simulink model "DBVF_2027"  (R2026b)
settings: Solver=ode4  StopTime=200  FixedStep=0.01
values from neighbouring files (symbols this model uses):
  Ah = 10    [model_workspace.m]
  all_written = 8191    [model_workspace.m]
  deg_to_cdeg = 100    [model_workspace.m]
  degE7 = 1.0E+7    (= 10000000)    [model_workspace.m]
  ground_elevation_m = 221    [model_workspace.m]
  I_0 = 0.31    [model_workspace.m]
  I_max = 100    [model_workspace.m]
  J_m = 8.6200e-04 * 1.5    (= 0.001293)    [model_workspace.m]
  K_e = 0.03080418253    [model_workspace.m]
  K_t = 0.03080418253    [model_workspace.m]
  K_u = 1    [model_workspace.m]
  m_to_cm = 100    [model_workspace.m]
  m_to_mm = 1000    [model_workspace.m]
  mps2_to_mG = 101.97    [model_workspace.m]
  n_cells = 6    [model_workspace.m]
  Pa_to_hPa = 0.01    [model_workspace.m]
  R_batt = 6*10e-4    (= 0.006)    [model_workspace.m]
  R_m = 0.17    [model_workspace.m]
  reference_location = [36.2071 -96.0102 221.3415]    [model_workspace.m]
  rho_kgpm3 = 1.225    [model_workspace.m]
  s_to_us = 1.0E+6    (= 1000000)    [model_workspace.m]
  timestep = 0.005    [model_workspace.m]
  uT_to_gauss = 0.01    [model_workspace.m]
undefined symbols (not defined in the file or in its folder): fractalcoef, Payload
libraries: uavmavlinklib x10, aerolibatmos2 x2, aerolibutil x2, simulink x2, aerolibasang x1, aerolibconvert2 x1, mspsensorlib x1, sharedtransform x1, sensorgpslib x1
settings Model: Creator=Teama  LastModifiedBy=Teama

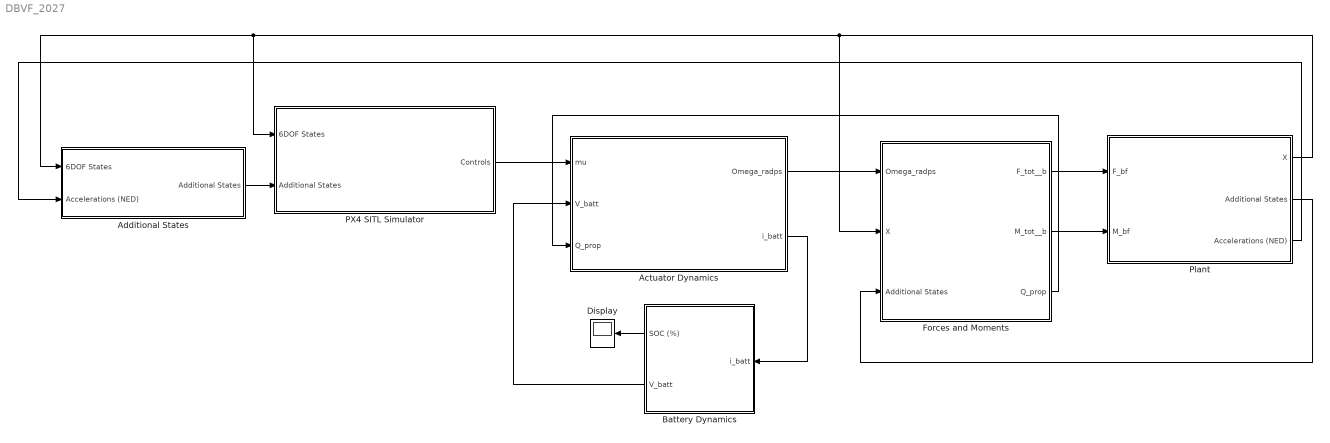
== system DBVF_2027 ==
  Actuator Dynamics : Subsystem
  Additional States : Subsystem
  Battery Dynamics : Subsystem
  Display : Display
  Forces and Moments : Subsystem
  PX4 SITL Simulator : Subsystem
  Plant : Subsystem
  wires:
  Actuator Dynamics/1(Omega_radps) -> Forces and Moments/1(Omega_radps)
  Actuator Dynamics/2(i_batt) -> Battery Dynamics/1(i_batt)
  Battery Dynamics/2(V_batt) -> Actuator Dynamics/2(V_batt)
  Forces and Moments/3(Q_prop) -> Actuator Dynamics/3(Q_prop)
  Additional States/1(Additional States) -> PX4 SITL Simulator/2(Additional States)
  PX4 SITL Simulator/1(Controls) -> Actuator Dynamics/1(mu)
  Battery Dynamics/1(SOC (%)) -> Display/1
  Plant/1(X) -> Forces and Moments/2(X), PX4 SITL Simulator/1(6DOF States), Additional States/1(6DOF States)
  Forces and Moments/1(F_tot__b) -> Plant/1(F_bf)
  Forces and Moments/2(M_tot__b) -> Plant/2(M_bf)
  Plant/2(Additional States) -> Forces and Moments/3(Additional States)
  Plant/3(Accelerations (NED)) -> Additional States/2(Accelerations (NED))

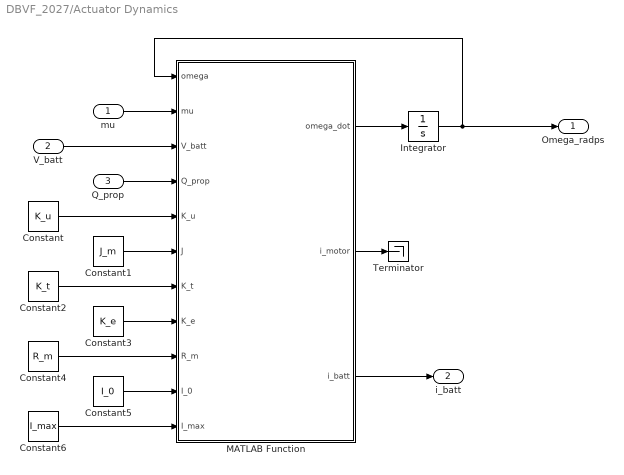
== system DBVF_2027/Actuator Dynamics ==
  mu : Inport
  V_batt : Inport  Port=2
  Q_prop : Inport  Port=3
  Constant : Constant  Value=K_u
  Constant1 : Constant  Value=J_m
  Constant2 : Constant  Value=K_t
  Constant3 : Constant  Value=K_e
  Constant4 : Constant  Value=R_m
  Constant5 : Constant  Value=I_0
  Constant6 : Constant  Value=I_max
  Integrator : Integrator
  MATLAB Function : MATLAB Function  TreatAsAtomicUnit=on
  Terminator : Terminator
  Omega_radps : Outport
  i_batt : Outport  Port=2
  wires:
  mu/1 -> MATLAB Function/2(mu)
  MATLAB Function/1(omega_dot) -> Integrator/1
  Integrator/1 -> MATLAB Function/1(omega), Omega_radps/1
  V_batt/1 -> MATLAB Function/3(V_batt)
  Q_prop/1 -> MATLAB Function/4(Q_prop)
  MATLAB Function/2(i_motor) -> Terminator/1
  MATLAB Function/3(i_batt) -> i_batt/1
  Constant/1 -> MATLAB Function/5(K_u)
  Constant1/1 -> MATLAB Function/6(J)
  Constant2/1 -> MATLAB Function/7(K_t)
  Constant3/1 -> MATLAB Function/8(K_e)
  Constant4/1 -> MATLAB Function/9(R_m)
  Constant5/1 -> MATLAB Function/10(I_0)
  Constant6/1 -> MATLAB Function/11(I_max)

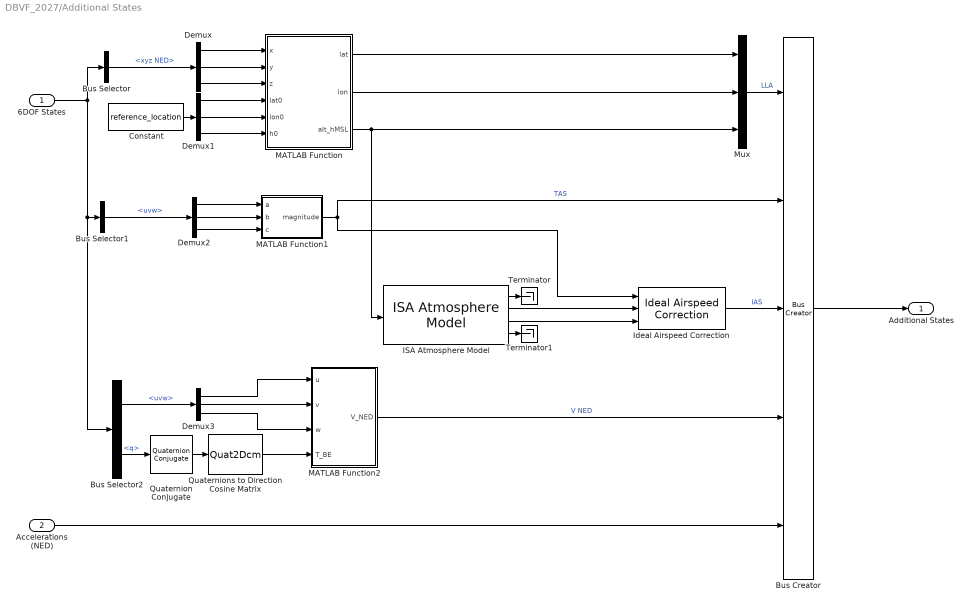
== system DBVF_2027/Additional States ==
  6DOF States : Inport
  Accelerations (NED) : Inport  Port=2
  Bus Creator : BusCreator  Inputs=5
  Bus Selector : BusSelector  OutputSignals=xyz NED
  Bus Selector1 : BusSelector  OutputSignals=uvw
  Bus Selector2 : BusSelector  OutputSignals=uvw,q
  Constant : Constant  Value=reference_location
  Demux{,1..3} (4 alike) : Demux  Outputs=3
  ISA Atmosphere Model : aerolibatmos2/ISA Atmosphere Model  useExtended=off  action=None  custom=off  viscosityOut=off  g=9.80665  gamma=1.4  R=287.0531  L=0.0065  h_trop=11000  h_strat=20000  rho0=1.225  P0=101325  T0=288.15  h0=0  S=110.4  Tref=273.15  muref=1.716e-5
  Ideal Airspeed Correction : aerolibasang/Ideal Airspeed Correction  units=Metric (MKS)  vel_in=TAS  vel_out_tas=CAS  vel_out_eas=TAS  vel_out_cas=TAS  method=Table Lookup  SubOnly=off  action=None
  MATLAB Function : MATLAB Function  TreatAsAtomicUnit=on
  MATLAB Function1 : MATLAB Function  TreatAsAtomicUnit=on
  MATLAB Function2 : MATLAB Function  TreatAsAtomicUnit=on
  Mux : Mux  Inputs=3
  Quaternion Conjugate : aerolibutil/Quaternion Conjugate
  Quaternions to Direction Cosine Matrix : Quat2Dcm
  Terminator : Terminator
  Terminator1 : Terminator
  Additional States : Outport
  wires:
  Bus Creator/1 -> Additional States/1
  6DOF States/1 -> Bus Selector2/1, Bus Selector1/1, Bus Selector/1
  Bus Selector/1 -> Demux/1  "<xyz NED>"
  MATLAB Function/1(lat) -> Mux/1
  MATLAB Function/2(lon) -> Mux/2
  MATLAB Function/3(alt_hMSL) -> Mux/3, ISA Atmosphere Model/1
  Mux/1 -> Bus Creator/1  "LLA"
  Demux/1 -> MATLAB Function/1(x)
  Demux/2 -> MATLAB Function/2(y)
  Demux/3 -> MATLAB Function/3(z)
  Constant/1 -> Demux1/1
  Demux1/1 -> MATLAB Function/4(lat0)
  Demux1/2 -> MATLAB Function/5(lon0)
  Demux1/3 -> MATLAB Function/6(h0)
  Ideal Airspeed Correction/1 -> Bus Creator/3  "IAS"
  Bus Selector1/1 -> Demux2/1  "<uvw>"
  Demux2/1 -> MATLAB Function1/1(a)
  Demux2/2 -> MATLAB Function1/2(b)
  Demux2/3 -> MATLAB Function1/3(c)
  MATLAB Function1/1(magnitude) -> Ideal Airspeed Correction/1, Bus Creator/2  "TAS"
  ISA Atmosphere Model/3 -> Ideal Airspeed Correction/3
  ISA Atmosphere Model/2 -> Ideal Airspeed Correction/2
  ISA Atmosphere Model/1 -> Terminator/1
  ISA Atmosphere Model/4 -> Terminator1/1
  Quaternions to Direction Cosine Matrix/1 -> MATLAB Function2/4(T_BE)
  Bus Selector2/1 -> Demux3/1  "<uvw>"
  Bus Selector2/2 -> Quaternion Conjugate/1  "<q>"
  Demux3/1 -> MATLAB Function2/1(u)
  Demux3/2 -> MATLAB Function2/2(v)
  Demux3/3 -> MATLAB Function2/3(w)
  MATLAB Function2/1(V_NED) -> Bus Creator/4  "V NED"
  Quaternion Conjugate/1 -> Quaternions to Direction Cosine Matrix/1
  Accelerations (NED)/1 -> Bus Creator/5

== system DBVF_2027/Battery Dynamics ==
  i_batt : Inport
  Constant : Constant  Value=Ah
  Constant1 : Constant  Value=R_batt
  Gain : Gain  Gain=n_cells
  Gain1 : Gain  Gain=100
  Integrator : Integrator
  LiPo Discharge Curve : Lookup_n-D  NumberOfTableDimensions=1  BreakpointsForDimension1="[0    0.05  0.10  0.20  0.30  0.40  0.50  0.60  0.70  0.80  0.90  1.00]"  Table="[3.20 3.45  3.55  3.65  3.70  3.74  3.77  3.80  3.84  3.90  4.00  4.20]"  InternalRulePriority=Speed  RndMeth=Simplest
  battery dynamics wrapper : MATLAB Function  TreatAsAtomicUnit=on
  SOC (%) : Outport
  V_batt : Outport  Port=2
  wires:
  i_batt/1 -> battery dynamics wrapper/1(I_batt_in)
  battery dynamics wrapper/1(SOC_dot) -> Integrator/1
  Integrator/1 -> Gain1/1, LiPo Discharge Curve/1
  LiPo Discharge Curve/1 -> Gain/1
  Gain/1 -> battery dynamics wrapper/2(V_OC)
  battery dynamics wrapper/2(V_batt) -> V_batt/1
  Gain1/1 -> SOC (%)/1
  Constant/1 -> battery dynamics wrapper/4(Ah)
  Constant1/1 -> battery dynamics wrapper/3(R_batt)

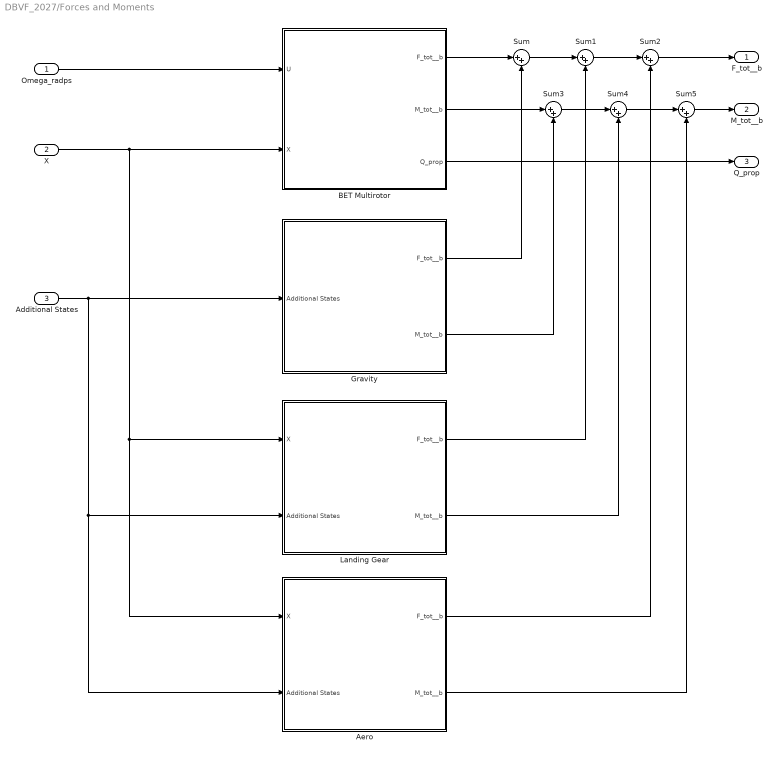
== system DBVF_2027/Forces and Moments ==
  Omega_radps : Inport
  X : Inport  Port=2
  Additional States : Inport  Port=3
  Aero : Subsystem
  BET Multirotor : Subsystem
  Gravity : Subsystem
  Landing Gear : Subsystem
  Sum{,1..5} (6 alike) : Sum  Inputs=|++
  F_tot__b : Outport
  M_tot__b : Outport  Port=2
  Q_prop : Outport  Port=3
  wires:
  Omega_radps/1 -> BET Multirotor/1(U)
  X/1 -> Landing Gear/1(X), Aero/1(X), BET Multirotor/2(X)
  Additional States/1 -> Landing Gear/2(Additional States), Aero/2(Additional States), Gravity/1(Additional States)
  BET Multirotor/1(F_tot__b) -> Sum/1
  Gravity/1(F_tot__b) -> Sum/2
  Sum/1 -> Sum1/1
  Aero/1(F_tot__b) -> Sum2/2
  Sum1/1 -> Sum2/1
  Sum2/1 -> F_tot__b/1
  BET Multirotor/2(M_tot__b) -> Sum3/1
  Gravity/2(M_tot__b) -> Sum3/2
  Sum3/1 -> Sum4/1
  Sum5/1 -> M_tot__b/1
  Sum4/1 -> Sum5/1
  Aero/2(M_tot__b) -> Sum5/2
  BET Multirotor/3(Q_prop) -> Q_prop/1
  Landing Gear/1(F_tot__b) -> Sum1/2
  Landing Gear/2(M_tot__b) -> Sum4/2

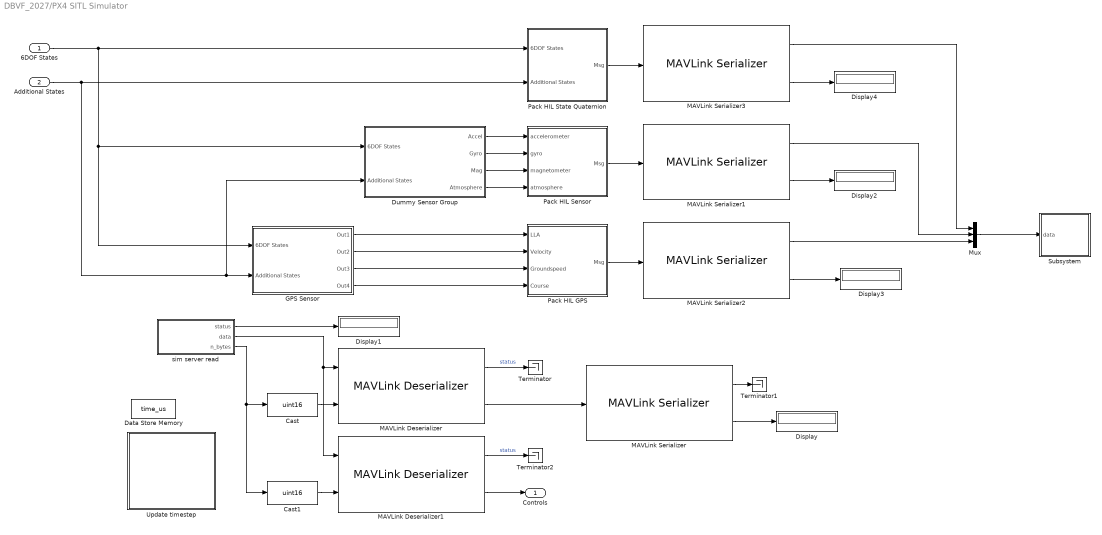
== system DBVF_2027/PX4 SITL Simulator ==
  6DOF States : Inport
  Additional States : Inport  Port=2
  Cast : DataTypeConversion  OutDataTypeStr=uint16  SaturateOnIntegerOverflow=off  RndMeth=Floor
  Cast1 : DataTypeConversion  OutDataTypeStr=uint16  SaturateOnIntegerOverflow=off  RndMeth=Floor
  Data Store Memory : DataStoreMemory  DataStoreName=time_us  WriteAfterWriteMsg=warning  ShowAdditionalParam=off  OutDataTypeStr=uint64
  Display{,1..4} (5 alike) : Display
  Dummy Sensor Group : Subsystem
  GPS Sensor : Subsystem
  MAVLink Deserializer : uavmavlinklib/MAVLink Deserializer  dialectSource=Select from standard MAVLink dialects  dialect=common.xml  dialectCustom=common.xml  version=2  messageType=HEARTBEAT  inputDataLength=on  SystemIDFilter=off  systemID=1  ComponentIDFilter=off  componentID=1  queueMsg=off  queueMsgSize=50  dropNum=off
  MAVLink Deserializer1 : uavmavlinklib/MAVLink Deserializer  dialectSource=Select from standard MAVLink dialects  dialect=common.xml  dialectCustom=common.xml  version=2  messageType=HIL_ACTUATOR_CONTROLS  inputDataLength=on  SystemIDFilter=off  systemID=1  ComponentIDFilter=off  componentID=1  queueMsg=off  queueMsgSize=50  dropNum=off
  MAVLink Serializer : uavmavlinklib/MAVLink Serializer  dialectSource=Select from standard MAVLink dialects  dialect=common.xml  dialectCustom=common.xml  version=2  messageType=HEARTBEAT
  MAVLink Serializer1 : uavmavlinklib/MAVLink Serializer  dialectSource=Select from standard MAVLink dialects  dialect=common.xml  dialectCustom=common.xml  version=2  messageType=HIL_SENSOR
  MAVLink Serializer2 : uavmavlinklib/MAVLink Serializer  dialectSource=Select from standard MAVLink dialects  dialect=common.xml  dialectCustom=common.xml  version=2  messageType=HIL_GPS
  MAVLink Serializer3 : uavmavlinklib/MAVLink Serializer  dialectSource=Select from standard MAVLink dialects  dialect=common.xml  dialectCustom=common.xml  version=2  messageType=HIL_STATE_QUATERNION
  Mux : Mux  Inputs=3
  Pack HIL GPS : Subsystem
  Pack HIL Sensor : Subsystem
  Pack HIL State Quaternion : Subsystem
  Subsystem : Subsystem
  Terminator : Terminator
  Terminator1 : Terminator
  Terminator2 : Terminator
  Update timestep : Subsystem
  sim server read : MATLAB Function  TreatAsAtomicUnit=on
  Controls : Outport
  wires:
  sim server read/1(status) -> Display1/1
  MAVLink Serializer/1 -> Terminator1/1
  MAVLink Serializer3/1 -> Mux/1
  MAVLink Serializer3/2 -> Display4/1
  sim server read/2(data) -> MAVLink Deserializer1/1, MAVLink Deserializer/1
  Dummy Sensor Group/1(Accel) -> Pack HIL Sensor/1(accelerometer)
  Dummy Sensor Group/2(Gyro) -> Pack HIL Sensor/2(gyro)
  Dummy Sensor Group/4(Atmosphere) -> Pack HIL Sensor/4(atmosphere)
  Pack HIL State Quaternion/1(Msg) -> MAVLink Serializer3/1
  Dummy Sensor Group/3(Mag) -> Pack HIL Sensor/3(magnetometer)
  MAVLink Serializer1/1 -> Mux/2
  Additional States/1 -> Dummy Sensor Group/2(Additional States), GPS Sensor/2(Additional States), Pack HIL State Quaternion/2(Additional States)
  MAVLink Serializer2/2 -> Display3/1
  Pack HIL Sensor/1(Msg) -> MAVLink Serializer1/1
  MAVLink Serializer1/2 -> Display2/1
  MAVLink Serializer2/1 -> Mux/3
  MAVLink Serializer/2 -> Display/1
  Pack HIL GPS/1(Msg) -> MAVLink Serializer2/1
  MAVLink Deserializer/1 -> Terminator/1  "status"
  MAVLink Deserializer/2 -> MAVLink Serializer/1
  6DOF States/1 -> GPS Sensor/1(6DOF States), Dummy Sensor Group/1(6DOF States), Pack HIL State Quaternion/1(6DOF States)
  MAVLink Deserializer1/1 -> Terminator2/1  "status"
  MAVLink Deserializer1/2 -> Controls/1
  Mux/1 -> Subsystem/1(data)
  GPS Sensor/1(Out1) -> Pack HIL GPS/1(LLA)
  GPS Sensor/2(Out2) -> Pack HIL GPS/2(Velocity)
  GPS Sensor/3(Out3) -> Pack HIL GPS/3(Groundspeed)
  GPS Sensor/4(Out4) -> Pack HIL GPS/4(Course)
  sim server read/3(n_bytes) -> Cast/1, Cast1/1
  Cast/1 -> MAVLink Deserializer/2
  Cast1/1 -> MAVLink Deserializer1/2

== system DBVF_2027/Plant ==
  F_bf : Inport
  M_bf : Inport  Port=2
  6DOF (Quaternion) : EOM6DOFBodyQuat  xme_0=[0 0 -ground_elevation_m]  mass_0=m_kg  inertia=I_kgm2  mass_flag=on
  A_bf to A_NED : Subsystem
  Bus Creator : BusCreator  Inputs=4
  Bus Creator1 : BusCreator  Inputs=4
  Terminator : Terminator
  X : Outport
  Additional States : Outport  Port=2
  Accelerations (NED) : Outport  Port=3
  wires:
  6DOF (Quaternion)/5 -> A_bf to A_NED/3(DCM_be), Bus Creator1/2  "DCM_be"
  6DOF (Quaternion)/1 -> Bus Creator1/1  "V_e"
  6DOF (Quaternion)/3 -> Terminator/1
  6DOF (Quaternion)/2 -> Bus Creator/1  "X_e"
  M_bf/1 -> 6DOF (Quaternion)/2
  6DOF (Quaternion)/7 -> Bus Creator/3  "Omega_b"
  6DOF (Quaternion)/6 -> Bus Creator/2  "V_b"
  6DOF (Quaternion)/4 -> Bus Creator/4  "q"
  F_bf/1 -> A_bf to A_NED/1(F_bf), 6DOF (Quaternion)/1
  Bus Creator/1 -> X/1
  Bus Creator1/1 -> Additional States/1
  6DOF (Quaternion)/8 -> A_bf to A_NED/2(m), Bus Creator1/3  "m"
  A_bf to A_NED/1(Accelerations (NED)) -> Accelerations (NED)/1
  6DOF (Quaternion)/9 -> Bus Creator1/4  "I"

== system DBVF_2027/Forces and Moments/Aero ==
  X : Inport
  Additional States : Inport  Port=2
  F_tot__b : Outport
  M_tot__b : Outport  Port=2
  wires:
  ? -> F_tot__b/1
  ? -> M_tot__b/1

== system DBVF_2027/Forces and Moments/BET Multirotor ==
  U : Inport
  X : Inport  Port=2
  Constant : Constant  Value=rho_kgpm3  VectorParams1D=off
  Multirotor : Multirotor  modelMode=With flap effects  CTCQMode=Compute using BEMT
  F_tot__b : Outport
  M_tot__b : Outport  Port=2
  Q_prop : Outport  Port=3
  wires:
  Multirotor/2 -> M_tot__b/1
  U/1 -> Multirotor/1
  X/1 -> ?
  Multirotor/1 -> F_tot__b/1
  Constant/1 -> Multirotor/2

== system DBVF_2027/Forces and Moments/Gravity ==
  Additional States : Inport
  Bus Selector : BusSelector  OutputSignals=m,DCM_be
  MATLAB Function : MATLAB Function  TreatAsAtomicUnit=on
  F_tot__b : Outport
  M_tot__b : Outport  Port=2
  wires:
  Bus Selector/2 -> MATLAB Function/2(DCM_be)  "<DCM_be>"
  Bus Selector/1 -> MATLAB Function/1(m)  "<m>"
  Additional States/1 -> Bus Selector/1
  MATLAB Function/1(F_tot__b) -> F_tot__b/1
  MATLAB Function/2(M_tot__b) -> M_tot__b/1

== system DBVF_2027/Forces and Moments/Landing Gear ==
  X : Inport
  Additional States : Inport  Port=2
  Bus Selector : BusSelector  OutputSignals=DCM_be,m
  Constant : Constant  Value=reference_location(3)
  Landing Gear Subsystem : Subsystem  ReferencedSubsystem=Landing_Gear_Subsystem
  F_tot__b : Outport
  M_tot__b : Outport  Port=2
  wires:
  X/1 -> Landing Gear Subsystem/1
  Landing Gear Subsystem/1 -> F_tot__b/1
  Landing Gear Subsystem/2 -> M_tot__b/1
  Additional States/1 -> Bus Selector/1
  Bus Selector/1 -> Landing Gear Subsystem/2  "<DCM_be>"
  Bus Selector/2 -> Landing Gear Subsystem/4  "<m>"
  Constant/1 -> Landing Gear Subsystem/3

== system DBVF_2027/PX4 SITL Simulator/Dummy Sensor Group ==
  6DOF States : Inport
  Additional States : Inport  Port=2
  Dummy Barometer Data : Subsystem
  Dummy IMU Data : Subsystem
  Accel : Outport
  Gyro : Outport  Port=2
  Mag : Outport  Port=3
  Atmosphere : Outport  Port=4
  wires:
  Dummy IMU Data/1(Accel) -> Accel/1
  Dummy IMU Data/2(Gyro) -> Gyro/1
  Dummy IMU Data/3(Mag) -> Mag/1
  Dummy Barometer Data/1(Out1) -> Atmosphere/1
  6DOF States/1 -> Dummy IMU Data/2(6DOF States)
  Additional States/1 -> Dummy IMU Data/1(Additional States), Dummy Barometer Data/1(Additional States)

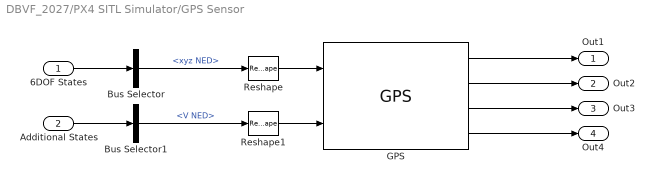
== system DBVF_2027/PX4 SITL Simulator/GPS Sensor ==
  6DOF States : Inport
  Additional States : Inport  Port=2
  Bus Selector : BusSelector  OutputSignals=xyz NED
  Bus Selector1 : BusSelector  OutputSignals=V NED
  GPS : sensorgpslib/GPS  DispRefFrame=NED  PositionInputFormat=Local  ReferenceLocation=reference_location  HorizontalPositionAccuracy=0.01  VerticalPositionAccuracy=0.01  VelocityAccuracy=0.01  DecayFactor=0.99  SeedDouble=67  SimulateUsing=Interpreted execution
      settings: LibrarySourceBlock=mspsensorlib/GPS
  Reshape : Reshape  OutputDimensionality=Row vector (2-D)
  Reshape1 : Reshape  OutputDimensionality=Row vector (2-D)
  Out1 : Outport
  Out2 : Outport  Port=2
  Out3 : Outport  Port=3
  Out4 : Outport  Port=4
  wires:
  Reshape/1 -> GPS/1
  GPS/1 -> Out1/1
  Reshape1/1 -> GPS/2
  Bus Selector/1 -> Reshape/1  "<xyz NED>"
  Bus Selector1/1 -> Reshape1/1  "<V NED>"
  GPS/4 -> Out4/1
  GPS/3 -> Out3/1
  GPS/2 -> Out2/1
  6DOF States/1 -> Bus Selector/1
  Additional States/1 -> Bus Selector1/1

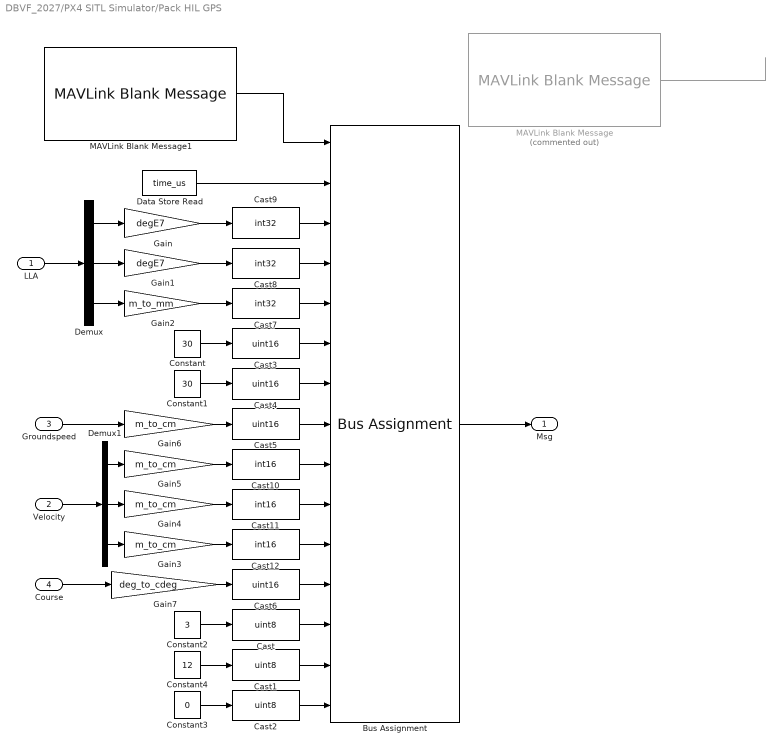
== system DBVF_2027/PX4 SITL Simulator/Pack HIL GPS ==
  LLA : Inport
  Velocity : Inport  Port=2
  Groundspeed : Inport  Port=3
  Course : Inport  Port=4
  Bus Assignment : BusAssignment  AssignedSignals=Payload.time_usec,Payload.lat,Payload.lon,Payload.alt,Payload.eph,Payload.epv,Payload.vel,Payload.vn,Payload.ve,Payload.vd,Payload.cog,Payload.fix_type,Payload.satellites_visible,Payload.id
  Cast : DataTypeConversion  OutDataTypeStr=uint8  SaturateOnIntegerOverflow=off  RndMeth=Floor
  Cast1 : DataTypeConversion  OutDataTypeStr=uint8  SaturateOnIntegerOverflow=off  RndMeth=Floor
  Cast10 : DataTypeConversion  OutDataTypeStr=int16  SaturateOnIntegerOverflow=off  RndMeth=Floor
  Cast11 : DataTypeConversion  OutDataTypeStr=int16  SaturateOnIntegerOverflow=off  RndMeth=Floor
  Cast12 : DataTypeConversion  OutDataTypeStr=int16  SaturateOnIntegerOverflow=off  RndMeth=Floor
  Cast2 : DataTypeConversion  OutDataTypeStr=uint8  SaturateOnIntegerOverflow=off  RndMeth=Floor
  Cast{3..6} (4 alike) : DataTypeConversion  OutDataTypeStr=uint16  SaturateOnIntegerOverflow=off  RndMeth=Floor
  Cast7 : DataTypeConversion  OutDataTypeStr=int32  SaturateOnIntegerOverflow=off  RndMeth=Floor
  Cast8 : DataTypeConversion  OutDataTypeStr=int32  SaturateOnIntegerOverflow=off  RndMeth=Floor
  Cast9 : DataTypeConversion  OutDataTypeStr=int32  SaturateOnIntegerOverflow=off  RndMeth=Floor
  Constant : Constant  Value=30
  Constant1 : Constant  Value=30  OutDataTypeStr=uint16
  Constant2 : Constant  Value=3
  Constant3 : Constant  Value=0
  Constant4 : Constant  Value=12
  Data Store Read : DataStoreRead  DataStoreName=time_us  IndexOptions=Index vector (dialog)  Indices=1  OutputSizes=1
  Demux : Demux  Outputs=3
  Demux1 : Demux  Outputs=3
  Gain : Gain  Gain=degE7
  Gain1 : Gain  Gain=degE7
  Gain2 : Gain  Gain=m_to_mm
  Gain{3..6} (4 alike) : Gain  Gain=m_to_cm
  Gain7 : Gain  Gain=deg_to_cdeg
  MAVLink Blank Message : uavmavlinklib/MAVLink Blank Message  Commented=on  dialectSource=Select from standard MAVLink dialects  dialect=common.xml  dialectCustom=common.xml  version=2  messageType=HIL_GPS  SystemID=2  ComponentID=51  SampleTime=timestep
  MAVLink Blank Message1 : uavmavlinklib/MAVLink Blank Message  dialectSource=Select from standard MAVLink dialects  dialect=common.xml  dialectCustom=common.xml  version=2  messageType=HIL_GPS  SystemID=1  ComponentID=51  SampleTime=timestep
  Msg : Outport
  wires:
  Bus Assignment/1 -> Msg/1
  Data Store Read/1 -> Bus Assignment/2
  MAVLink Blank Message/1 -> ?
  Demux/1 -> Gain/1
  Demux/2 -> Gain1/1
  Demux/3 -> Gain2/1
  Constant/1 -> Cast3/1
  Constant1/1 -> Cast4/1
  LLA/1 -> Demux/1
  Constant2/1 -> Cast/1
  Cast/1 -> Bus Assignment/13
  Constant3/1 -> Cast2/1
  Constant4/1 -> Cast1/1
  Cast1/1 -> Bus Assignment/14
  Cast2/1 -> Bus Assignment/15
  Cast3/1 -> Bus Assignment/6
  Cast4/1 -> Bus Assignment/7
  Groundspeed/1 -> Gain6/1
  Cast5/1 -> Bus Assignment/8
  Velocity/1 -> Demux1/1
  Demux1/1 -> Gain5/1
  Demux1/2 -> Gain4/1
  Demux1/3 -> Gain3/1
  Cast6/1 -> Bus Assignment/12
  Course/1 -> Gain7/1
  Gain/1 -> Cast9/1
  Gain1/1 -> Cast8/1
  Gain2/1 -> Cast7/1
  Cast7/1 -> Bus Assignment/5
  Cast8/1 -> Bus Assignment/4
  Cast9/1 -> Bus Assignment/3
  Cast10/1 -> Bus Assignment/9
  Cast11/1 -> Bus Assignment/10
  Cast12/1 -> Bus Assignment/11
  Gain3/1 -> Cast12/1
  Gain4/1 -> Cast11/1
  Gain5/1 -> Cast10/1
  Gain6/1 -> Cast5/1
  Gain7/1 -> Cast6/1
  MAVLink Blank Message1/1 -> Bus Assignment/1

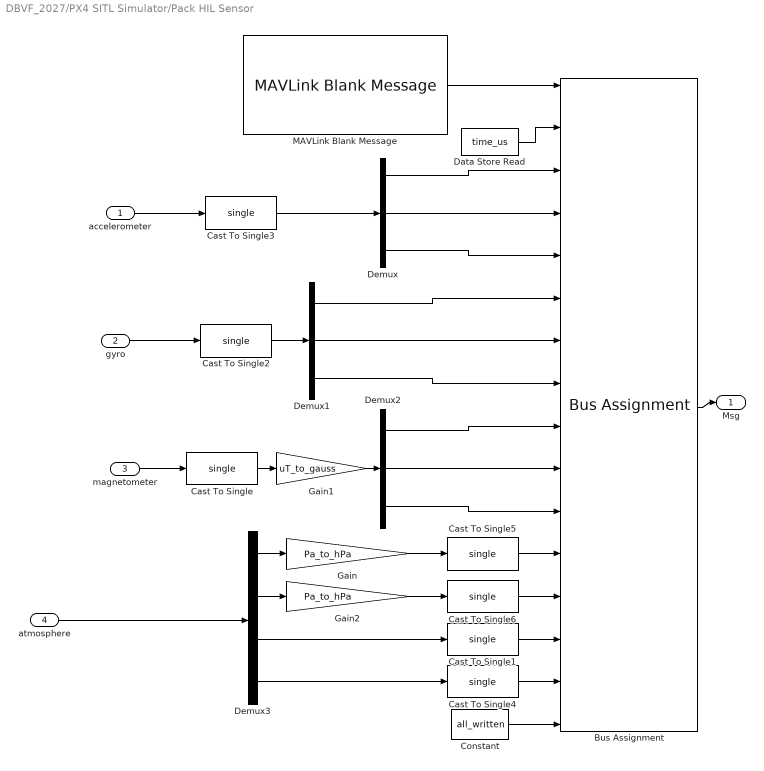
== system DBVF_2027/PX4 SITL Simulator/Pack HIL Sensor ==
  accelerometer : Inport
  gyro : Inport  Port=2
  magnetometer : Inport  Port=3
  atmosphere : Inport  Port=4
  Bus Assignment : BusAssignment  AssignedSignals=Payload.time_usec,Payload.xacc,Payload.yacc,Payload.zacc,Payload.xgyro,Payload.ygyro,Payload.zgyro,Payload.xmag,Payload.ymag,Payload.zmag,Payload.abs_pressure,Payload.diff_pressure,Payload.pressure_alt,Payload.temperature,Payload.fields_updated
  Cast To Single{,1..6} (7 alike) : DataTypeConversion  OutDataTypeStr=single  SaturateOnIntegerOverflow=off  RndMeth=Floor
  Constant : Constant  Value=all_written  OutDataTypeStr=uint32
  Data Store Read : DataStoreRead  DataStoreName=time_us  IndexOptions=Index vector (dialog)  Indices=1  OutputSizes=1
  Demux : Demux  Outputs=3
  Demux1 : Demux  Outputs=3
  Demux2 : Demux  Outputs=3
  Demux3 : Demux
  Gain : Gain  Gain=Pa_to_hPa
  Gain1 : Gain  Gain=uT_to_gauss
  Gain2 : Gain  Gain=Pa_to_hPa
  MAVLink Blank Message : uavmavlinklib/MAVLink Blank Message  dialectSource=Select from standard MAVLink dialects  dialect=common.xml  dialectCustom=common.xml  version=2  messageType=HIL_SENSOR  SystemID=2  ComponentID=51  SampleTime=timestep
  Msg : Outport
  wires:
  gyro/1 -> Cast To Single2/1
  Demux1/3 -> Bus Assignment/8
  Demux1/1 -> Bus Assignment/6
  MAVLink Blank Message/1 -> Bus Assignment/1
  Demux/3 -> Bus Assignment/5
  Data Store Read/1 -> Bus Assignment/2
  Demux/1 -> Bus Assignment/3
  Demux1/2 -> Bus Assignment/7
  Bus Assignment/1 -> Msg/1
  Demux/2 -> Bus Assignment/4
  Demux2/1 -> Bus Assignment/9
  Demux2/2 -> Bus Assignment/10
  Demux2/3 -> Bus Assignment/11
  Demux3/1 -> Gain/1
  Demux3/4 -> Cast To Single4/1
  Demux3/2 -> Gain2/1
  magnetometer/1 -> Cast To Single/1
  accelerometer/1 -> Cast To Single3/1
  Cast To Single/1 -> Gain1/1
  atmosphere/1 -> Demux3/1
  Cast To Single2/1 -> Demux1/1
  Cast To Single3/1 -> Demux/1
  Gain1/1 -> Demux2/1
  Constant/1 -> Bus Assignment/16
  Gain/1 -> Cast To Single5/1
  Demux3/3 -> Cast To Single1/1
  Cast To Single4/1 -> Bus Assignment/15
  Cast To Single5/1 -> Bus Assignment/12
  Cast To Single1/1 -> Bus Assignment/14
  Gain2/1 -> Cast To Single6/1
  Cast To Single6/1 -> Bus Assignment/13

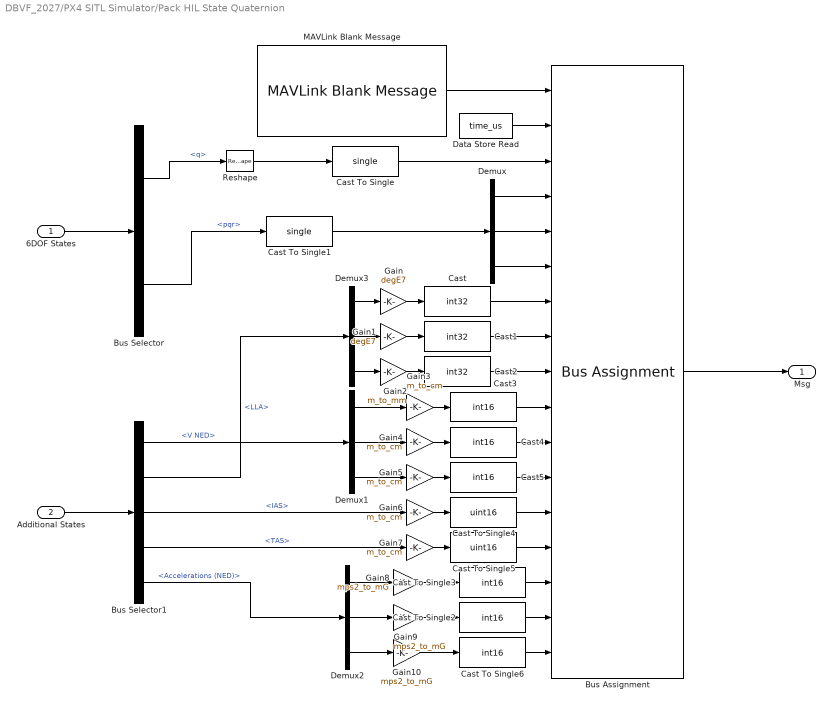
== system DBVF_2027/PX4 SITL Simulator/Pack HIL State Quaternion ==
  6DOF States : Inport
  Additional States : Inport  Port=2
  Bus Assignment : BusAssignment  AssignedSignals=Payload.time_usec,Payload.attitude_quaternion,Payload.rollspeed,Payload.pitchspeed,Payload.yawspeed,Payload.lat,Payload.lon,Payload.alt,Payload.vx,Payload.vy,Payload.vz,Payload.ind_airspeed,Payload.true_airspeed,Payload.xacc,Payload.yacc,Payload.zacc
  Bus Selector : BusSelector  OutputSignals=q,pqr
  Bus Selector1 : BusSelector  OutputSignals=V NED,LLA,IAS,TAS,Accelerations (NED)
  Cast : DataTypeConversion  OutDataTypeStr=int32  SaturateOnIntegerOverflow=off  RndMeth=Floor
  Cast To Single : DataTypeConversion  OutDataTypeStr=single  SaturateOnIntegerOverflow=off  RndMeth=Floor
  Cast To Single1 : DataTypeConversion  OutDataTypeStr=single  SaturateOnIntegerOverflow=off  RndMeth=Floor
  Cast To Single2 : DataTypeConversion  OutDataTypeStr=int16  SaturateOnIntegerOverflow=off  RndMeth=Floor
  Cast To Single3 : DataTypeConversion  OutDataTypeStr=int16  SaturateOnIntegerOverflow=off  RndMeth=Floor
  Cast To Single4 : DataTypeConversion  OutDataTypeStr=uint16  SaturateOnIntegerOverflow=off  RndMeth=Floor
  Cast To Single5 : DataTypeConversion  OutDataTypeStr=uint16  SaturateOnIntegerOverflow=off  RndMeth=Floor
  Cast To Single6 : DataTypeConversion  OutDataTypeStr=int16  SaturateOnIntegerOverflow=off  RndMeth=Floor
  Cast1 : DataTypeConversion  OutDataTypeStr=int32  SaturateOnIntegerOverflow=off  RndMeth=Floor
  Cast2 : DataTypeConversion  OutDataTypeStr=int32  SaturateOnIntegerOverflow=off  RndMeth=Floor
  Cast3 : DataTypeConversion  OutDataTypeStr=int16  SaturateOnIntegerOverflow=off  RndMeth=Floor
  Cast4 : DataTypeConversion  OutDataTypeStr=int16  SaturateOnIntegerOverflow=off  RndMeth=Floor
  Cast5 : DataTypeConversion  OutDataTypeStr=int16  SaturateOnIntegerOverflow=off  RndMeth=Floor
  Data Store Read : DataStoreRead  DataStoreName=time_us  IndexOptions=Index vector (dialog)  Indices=1  OutputSizes=1
  Demux{,1..3} (4 alike) : Demux  Outputs=3
  Gain : Gain  Gain=degE7
  Gain1 : Gain  Gain=degE7
  Gain10 : Gain  Gain=mps2_to_mG
  Gain2 : Gain  Gain=m_to_mm
  Gain{3..7} (5 alike) : Gain  Gain=m_to_cm
  Gain8 : Gain  Gain=mps2_to_mG
  Gain9 : Gain  Gain=mps2_to_mG
  MAVLink Blank Message : uavmavlinklib/MAVLink Blank Message  dialectSource=Select from standard MAVLink dialects  dialect=common.xml  dialectCustom=common.xml  version=2  messageType=HIL_STATE_QUATERNION  SystemID=2  ComponentID=51  SampleTime=timestep
  Reshape : Reshape  OutputDimensionality=Row vector (2-D)
  Msg : Outport
  wires:
  Bus Assignment/1 -> Msg/1
  Data Store Read/1 -> Bus Assignment/2
  MAVLink Blank Message/1 -> Bus Assignment/1
  6DOF States/1 -> Bus Selector/1
  Bus Selector/1 -> Reshape/1  "<q>"
  Cast To Single/1 -> Bus Assignment/3
  Bus Selector/2 -> Cast To Single1/1  "<pqr>"
  Cast To Single1/1 -> Demux/1
  Demux/1 -> Bus Assignment/4
  Demux/2 -> Bus Assignment/5
  Demux/3 -> Bus Assignment/6
  Demux1/2 -> Gain4/1
  Demux1/3 -> Gain5/1
  Demux1/1 -> Gain3/1
  Demux2/1 -> Gain8/1
  Demux2/2 -> Gain9/1
  Demux2/3 -> Gain10/1
  Additional States/1 -> Bus Selector1/1
  Bus Selector1/3 -> Gain6/1  "<IAS>"
  Bus Selector1/4 -> Gain7/1  "<TAS>"
  Bus Selector1/2 -> Demux3/1  "<LLA>"
  Demux3/1 -> Gain/1
  Demux3/2 -> Gain1/1
  Demux3/3 -> Gain2/1
  Gain/1 -> Cast/1
  Gain1/1 -> Cast1/1
  Gain2/1 -> Cast2/1
  Cast/1 -> Bus Assignment/7
  Cast1/1 -> Bus Assignment/8
  Cast2/1 -> Bus Assignment/9
  Gain3/1 -> Cast3/1
  Gain4/1 -> Cast4/1
  Gain5/1 -> Cast5/1
  Gain6/1 -> Cast To Single4/1
  Gain7/1 -> Cast To Single5/1
  Cast To Single4/1 -> Bus Assignment/13
  Cast To Single5/1 -> Bus Assignment/14
  Cast3/1 -> Bus Assignment/10
  Cast4/1 -> Bus Assignment/11
  Cast5/1 -> Bus Assignment/12
  Reshape/1 -> Cast To Single/1
  Bus Selector1/1 -> Demux1/1  "<V NED>"
  Cast To Single3/1 -> Bus Assignment/15
  Cast To Single2/1 -> Bus Assignment/16
  Cast To Single6/1 -> Bus Assignment/17
  Gain8/1 -> Cast To Single3/1
  Gain9/1 -> Cast To Single2/1
  Gain10/1 -> Cast To Single6/1
  Bus Selector1/5 -> Demux2/1  "<Accelerations (NED)>"

== system DBVF_2027/PX4 SITL Simulator/Subsystem ==
  data : Inport
  sim server write : MATLAB Function  TreatAsAtomicUnit=on
  wires:
  data/1 -> sim server write/1(data)

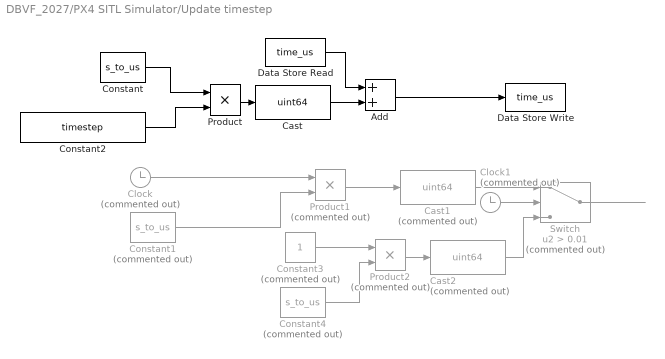
== system DBVF_2027/PX4 SITL Simulator/Update timestep ==
  Add : Sum
  Cast : DataTypeConversion  OutDataTypeStr=uint64  SaturateOnIntegerOverflow=off  RndMeth=Floor
  Cast1 : DataTypeConversion  Commented=on  OutDataTypeStr=uint64  SaturateOnIntegerOverflow=off  RndMeth=Floor
  Cast2 : DataTypeConversion  Commented=on  OutDataTypeStr=uint64  SaturateOnIntegerOverflow=off  RndMeth=Floor
  Clock : Clock  Commented=on
  Clock1 : Clock  Commented=on
  Constant : Constant  Value=s_to_us  OutDataTypeStr=uint64
  Constant1 : Constant  Commented=on  Value=s_to_us  OutDataTypeStr=uint64
  Constant2 : Constant  Value=timestep
  Constant3 : Constant  Commented=on
  Constant4 : Constant  Commented=on  Value=s_to_us  OutDataTypeStr=uint64
  Data Store Read : DataStoreRead  DataStoreName=time_us  IndexOptions=Index vector (dialog)  Indices=1  OutputSizes=1
  Data Store Write : DataStoreWrite  DataStoreName=time_us  IndexOptions=Index vector (dialog)  Indices=1  OutputSizes=1
  Product : Product
  Product1 : Product  Commented=on
  Product2 : Product  Commented=on
  Switch : Switch  Commented=on  Criteria=u2 > Threshold  Threshold=0.01  SaturateOnIntegerOverflow=off  InputSameDT=off
  wires:
  Constant/1 -> Product/1
  Data Store Read/1 -> Add/1
  Constant2/1 -> Product/2
  Product/1 -> Cast/1
  Cast/1 -> Add/2
  Add/1 -> Data Store Write/1
  Constant1/1 -> Product1/2
  Product1/1 -> Cast1/1
  Clock/1 -> Product1/1
  Cast1/1 -> Switch/1
  Clock1/1 -> Switch/2
  Switch/1 -> ?
  Constant3/1 -> Product2/1
  Constant4/1 -> Product2/2
  Product2/1 -> Cast2/1
  Cast2/1 -> Switch/3

== system DBVF_2027/Plant/A_bf to A_NED ==
  F_bf : Inport
  m : Inport  Port=2
  DCM_be : Inport  Port=3
  Divide : Product  Inputs=*/
  Invert 3x3 Matrix : aerolibutil/Invert  3x3 Matrix
  Matrix Multiply : Product  Multiplication=Matrix(*)
  Accelerations (NED) : Outport
  wires:
  m/1 -> Divide/2
  F_bf/1 -> Divide/1
  DCM_be/1 -> Invert 3x3 Matrix/1
  Invert 3x3 Matrix/1 -> Matrix Multiply/1
  Matrix Multiply/1 -> Accelerations (NED)/1
  Divide/1 -> Matrix Multiply/2  "a_bf"

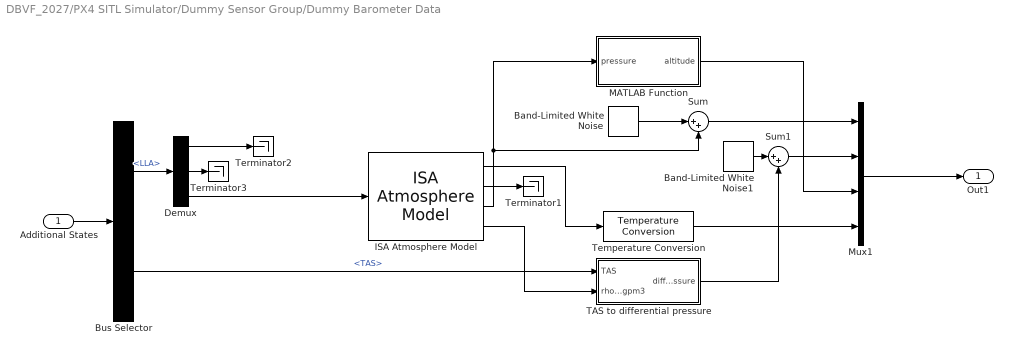
== system DBVF_2027/PX4 SITL Simulator/Dummy Sensor Group/Dummy Barometer Data ==
  Additional States : Inport
  Band-Limited White Noise : simulink/Sources/Band-Limited White Noise  Cov=[0.1]  Ts=timestep  seed=[23341]
  Band-Limited White Noise1 : simulink/Sources/Band-Limited White Noise  Cov=[0.1]  Ts=timestep  seed=[23341]
  Bus Selector : BusSelector  OutputSignals=LLA,TAS
  Demux : Demux  Outputs=3
  ISA Atmosphere Model : aerolibatmos2/ISA Atmosphere Model  useExtended=off  action=None  custom=off  viscosityOut=off  g=9.80665  gamma=1.4  R=287.0531  L=0.0065  h_trop=11000  h_strat=20000  rho0=1.225  P0=101325  T0=288.15  h0=0  S=110.4  Tref=273.15  muref=1.716e-5
  MATLAB Function : MATLAB Function  TreatAsAtomicUnit=on
  Mux1 : Mux
  Sum : Sum  Inputs=|++
  Sum1 : Sum  Inputs=|++
  TAS to differential pressure : MATLAB Function  TreatAsAtomicUnit=on
  Temperature Conversion : aerolibconvert2/Temperature Conversion  IU=K  OU=C
  Terminator1 : Terminator
  Terminator2 : Terminator
  Terminator3 : Terminator
  Out1 : Outport
  wires:
  ISA Atmosphere Model/4 -> TAS to differential pressure/2(rho_kgpm3)
  MATLAB Function/1(altitude) -> Mux1/3
  Temperature Conversion/1 -> Mux1/4
  ISA Atmosphere Model/3 -> Sum/2, MATLAB Function/1(pressure)
  ISA Atmosphere Model/1 -> Temperature Conversion/1
  Bus Selector/2 -> TAS to differential pressure/1(TAS)  "<TAS>"
  ISA Atmosphere Model/2 -> Terminator1/1
  Mux1/1 -> Out1/1
  Band-Limited White Noise/1 -> Sum/1
  Sum/1 -> Mux1/1
  Additional States/1 -> Bus Selector/1
  Bus Selector/1 -> Demux/1  "<LLA>"
  Demux/1 -> Terminator2/1
  Demux/2 -> Terminator3/1
  TAS to differential pressure/1(diff_pressure) -> Sum1/2
  Sum1/1 -> Mux1/2
  Band-Limited White Noise1/1 -> Sum1/1
  Demux/3 -> ISA Atmosphere Model/1

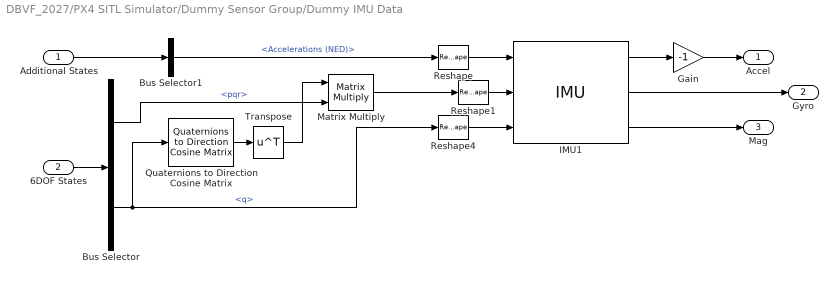
== system DBVF_2027/PX4 SITL Simulator/Dummy Sensor Group/Dummy IMU Data ==
  Additional States : Inport
  6DOF States : Inport  Port=2
  Bus Selector : BusSelector  OutputSignals=pqr,q
  Bus Selector1 : BusSelector  OutputSignals=Accelerations (NED)
  Gain : Gain  Gain=-1
  IMU1 : mspsensorlib/IMU  DispRefFrame=NED  TemperaturePort=off  Temperature=25  MagneticFieldPort=off  MagneticFieldNED=[ 21.5 1.16 43.1 ]  MagneticFieldENU=[ -2.4169, 27.5550, 16.0849 ]  SeedDouble=87254  SimulateUsing=Interpreted execution  AccelParamsMeasurementRange=Inf  AccelParamsResolution=0  AccelParamsConstantBias=[ 0, 0, 0 ]  AccelParamsAxesMisalignment=[ 0, 0, 0 ]  AccelParamsNoiseDensity=[ 0, 0, 0 ]  AccelParamsBiasInstability=[ 0, 0, 0 ]  AccelParamsBiasInstabilityNumerator=fractalcoef().Numerator  AccelParamsBiasInstabilityDenominator=fractalcoef().Denominator  AccelParamsRandomWalk=[ 0, 0, 0 ]  AccelParamsNoiseType=single-sided  AccelParamsTemperatureBias=[ 0, 0, 0 ]  AccelParamsTemperatureScaleFactor=[ 0, 0, 0 ]  GyroParamsMeasurementRange=Inf  GyroParamsResolution=0  GyroParamsConstantBias=[ 0, 0, 0 ]  GyroParamsAxesMisalignment=[ 0, 0, 0 ]  GyroParamsAccelerationBias=[ 0, 0, 0 ]  GyroParamsNoiseDensity=[ 0, 0, 0 ]  GyroParamsBiasInstability=[ 0, 0, 0 ]  GyroParamsBiasInstabilityNumerator=fractalcoef().Numerator  GyroParamsBiasInstabilityDenominator=fractalcoef().Denominator  GyroParamsRandomWalk=[ 0, 0, 0 ]  GyroParamsNoiseType=double-sided  GyroParamsTemperatureBias=[ 0, 0, 0 ]  GyroParamsTemperatureScaleFactor=[ 0, 0, 0 ]  MagParamsMeasurementRange=Inf  MagParamsResolution=0  MagParamsConstantBias=[ 0, 0, 0 ]  MagParamsAxesMisalignment=[ 0, 0, 0 ]  MagParamsNoiseDensity=0.0005  MagParamsBiasInstability=[ 0, 0, 0 ]  MagParamsBiasInstabilityNumerator=fractalcoef().Numerator  MagParamsBiasInstabilityDenominator=fractalcoef().Denominator  MagParamsRandomWalk=[ 0, 0, 0 ]  MagParamsNoiseType=double-sided  MagParamsTemperatureBias=[ 0, 0, 0 ]  MagParamsTemperatureScaleFactor=[ 0, 0, 0 ]
  Matrix Multiply : Product  Multiplication=Matrix(*)
  Quaternions to Direction Cosine Matrix : sharedtransform/Quaternions to  Direction Cosine Matrix  aMode=aMode
      settings: LibrarySourceBlock=|
      | aerolibtransform2/Quaternions to
      | Direction Cosine Matrix
  Reshape : Reshape  OutputDimensionality=Row vector (2-D)
  Reshape1 : Reshape  OutputDimensionality=Row vector (2-D)
  Reshape4 : Reshape  OutputDimensionality=Row vector (2-D)
  Transpose : Math  Operator=transpose
  Accel : Outport
  Gyro : Outport  Port=2
  Mag : Outport  Port=3
  wires:
  Reshape4/1 -> IMU1/3
  IMU1/1 -> Gain/1
  Gain/1 -> Accel/1
  IMU1/2 -> Gyro/1
  IMU1/3 -> Mag/1
  6DOF States/1 -> Bus Selector/1
  Bus Selector/1 -> Matrix Multiply/2  "<pqr>"
  Bus Selector/2 -> Quaternions to Direction Cosine Matrix/1, Reshape4/1  "<q>"
  Reshape/1 -> IMU1/1
  Reshape1/1 -> IMU1/2
  Quaternions to Direction Cosine Matrix/1 -> Transpose/1
  Transpose/1 -> Matrix Multiply/1
  Matrix Multiply/1 -> Reshape1/1
  Additional States/1 -> Bus Selector1/1
  Bus Selector1/1 -> Reshape/1  "<Accelerations (NED)>"

== matlab function DBVF_2027/PX4 SITL Simulator/Subsystem/sim server write ==
  data: data input
function fcn(data)

    coder.extrinsic('tcp_sim_server');
    
    tcp_sim_server("write", data);
end

== matlab function DBVF_2027/PX4 SITL Simulator/sim server read ==
  data: status output; data output; n_bytes output
function [status, data, n_bytes] = fcn()

    coder.extrinsic('tcp_sim_server');

    status = false;
    data = zeros(1,126,'uint8');
    n_bytes = 0;

    [status,data,n_bytes] = tcp_sim_server("read");
end

== matlab function DBVF_2027/Battery Dynamics/battery dynamics wrapper ==
  data: I_batt_in input; SOC_dot output; V_OC input; R_batt input; Ah input; V_batt output
function [SOC_dot, V_batt] = battery_dynamics_wrapper(I_batt_in, V_OC, R_batt, Ah)
    % initialize outputs
    I_batt_out = 0;
    V_batt = 0;
    P_batt = 0;
    SOC_dot = 0;

    [SOC_dot, V_batt] = battery_dynamics(I_batt_in, V_OC, R_batt, Ah);
end

== matlab function DBVF_2027/Actuator Dynamics/MATLAB Function ==
  data: omega input; mu input; omega_dot output; V_batt input; Q_prop input; K_u input; J input; K_t input; K_e input; R_m input; I_0 input; I_max input; i_motor output; i_batt output
function[omega_dot, i_motor, i_batt] = motor_dynamics_wrapper(omega, mu, V_batt, Q_prop, K_u, J, K_t, K_e, R_m, I_0, I_max)
    omega_dot = zeros(4,1);
    i_motor = zeros(4,1);
    i_batt = 0;

    [omega_dot, i_motor, i_batt] = motor_dynamics(mu, omega, V_batt, Q_prop, K_u, J, K_t, K_e, R_m, I_0, I_max);
end

== matlab function DBVF_2027/Additional States/MATLAB Function ==
  data: x input; lat output; y input; z input; lat0 input; lon0 input; h0 input; lon output; alt_hMSL output
function [lat, lon, alt_hMSL] = fcn(x, y, z, lat0, lon0, h0)
    [lat, lon, alt_hMSL] = ned2geodetic(x, y, z, lat0, lon0, h0, wgs84Ellipsoid);
end

== matlab function DBVF_2027/Additional States/MATLAB Function1 ==
  data: a input; magnitude output; b input; c input
function magnitude = fcn(a, b, c)
    magnitude = sqrt(a.^2 + b.^2 + c.^2);
end

== matlab function DBVF_2027/Forces and Moments/Gravity/MATLAB Function ==
  data: m input; F_tot__b output double size=[3,1]; M_tot__b output double size=[3,1]; DCM_be input
function [F_tot__b, M_tot__b] = gravity_wrapper(m, DCM_be)
    F_tot__b = zeros(3,1);
    M_tot__b = zeros(3,1);

    [F_tot__b, M_tot__b] = gravity(m, DCM_be);
end

== matlab function DBVF_2027/Additional States/MATLAB Function2 ==
  data: u input; V_NED output; v input; w input; T_BE input
function V_NED = fcn(u, v, w, T_BE)
    V_NED = T_BE * [u; v; w];
end

== matlab function DBVF_2027/PX4 SITL Simulator/Dummy Sensor Group/Dummy Barometer Data/MATLAB Function ==
  data: pressure input; altitude output
function altitude = fcn(pressure)
    altitude = 0;
    coder.extrinsic('atmospalt');
    altitude = atmospalt(pressure);
end

== matlab function DBVF_2027/PX4 SITL Simulator/Dummy Sensor Group/Dummy Barometer Data/TAS to differential pressure ==
  data: TAS input; diff_pressure output; rho_kgpm3 input
function diff_pressure = fcn(TAS, rho_kgpm3)
    diff_pressure = 0.5 * rho_kgpm3 * TAS^2;
end
